simulink model "AvonGasTurbineDgTwin"  (R2024b)
settings: Solver=VariableStepAuto  StartTime=0  StopTime=7200  FixedStep=1  RelTol=1e-3  EnableMultiTasking=on
InitFcn:
  | warning off
undefined symbols (not defined in the file or in its folder): ENV_ambient_moisture_pct, ENV_comp_inlet_press_kPa, ENV_comp_inlet_temp_C, ENV_FG_pressure_kPa, ENV_FG_temp_C
libraries: slpidlib x3, simulink x2
(part 2 of 3)

== system AvonGasTurbineDgTwin/FAULT_06_IGVStuck ==
  IGV Pos : Inport
  FAULT_06_multiplier : FromWorkspace  VariableName=FAULT_06_multiplier  SampleTime=-1
  Mux : Mux  Inputs=2
  Product : Product
  Scope{,1..3} (4 alike) : Scope  Commented=on
  Out1 : Outport
  wires:
  FAULT_06_multiplier/1 -> Product/1, Scope/1
  IGV Pos/1 -> Scope1/1, Mux/2, Product/2
  Product/1 -> Mux/1, Scope2/1, Out1/1
  Mux/1 -> Scope3/1

== system AvonGasTurbineDgTwin/FAULT_15_FuelPressReg ==
  In1 : Inport
  FAULT_15_multiplier : FromWorkspace  VariableName=FAULT_15_multiplier  SampleTime=-1
  Mux : Mux  Inputs=2
  Product : Product
  Scope{,1..3} (4 alike) : Scope  Commented=on
  Out1 : Outport
  wires:
  FAULT_15_multiplier/1 -> Product/1, Scope/1
  In1/1 -> Scope1/1, Mux/2, Product/2
  Product/1 -> Mux/1, Scope2/1, Out1/1
  Mux/1 -> Scope3/1

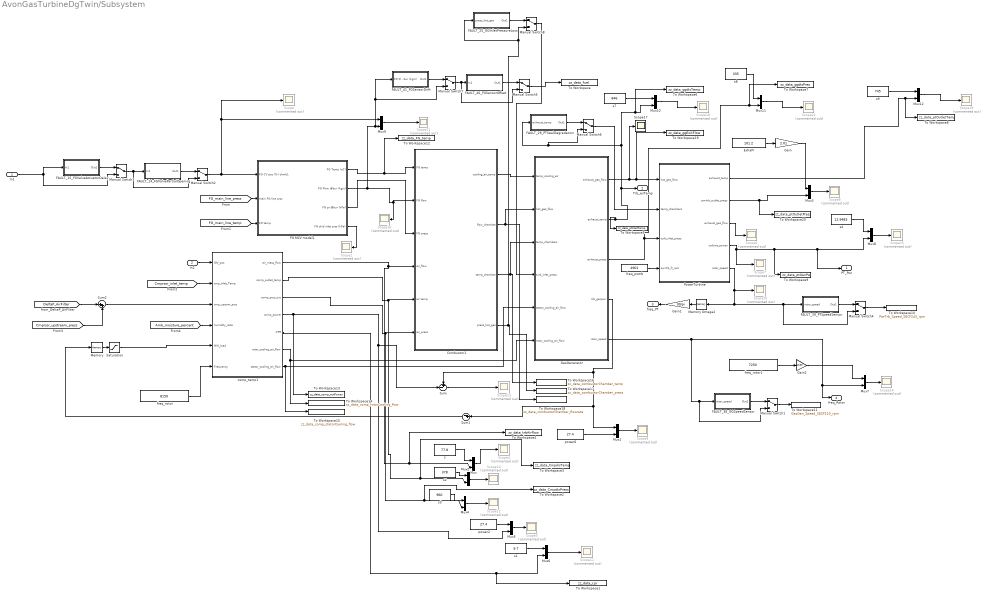
== system AvonGasTurbineDgTwin/Subsystem ==
  In1 : Inport
  In2 : Inport  Port=2
  Combustor1 : Subsystem
  ExhaPr : Constant  Value=101.2
  FAULT_14_FGValvePartialOpening : Subsystem
  FAULT_15_FGValveActuatorDelay : Subsystem
  FAULT_25_GGInletPressureLoss : Subsystem
  FAULT_29_PTSealDegradation : Subsystem
  FAULT_38_GGSpeedSensor : Subsystem
  FAULT_39_PTSpeedSensor : Subsystem
  FAULT_40_FGSensorOffset : Subsystem
  FAULT_41_FGSensorDrift : Subsystem
  FG MCV model1 : Subsystem
  Gain : Gain  Gain=2.01
  Gain1 : Gain  Gain=30/pi
  Gain2 : Gain  Gain=pi/30
  GasGenerator : Subsystem
  Manual Switch{1..8} (8 alike) : ManualSwitch
  Memory : Memory  InitialCondition=28.945
  Memory Omega2 : Memory  InitialCondition=pi/30*4901
  Mux{,1..12} (13 alike) : Mux  Inputs=2
  PowerTurbine : Subsystem
  Saturation : Saturate  UpperLimit=40  LowerLimit=1
  Scope{,2..4,6..16,18..22} (20 alike) : Scope  Commented=on
  Scope17 : Scope
  Sum : Sum  Inputs=+-|
  Sum1 : Sum  Inputs=-+|
  Sum2 : Sum  Inputs=|++
  To Workspace : ToWorkspace  VariableName=zz_data_fuel  SampleTime=0.2
  To Workspace1 : ToWorkspace  VariableName=zz_data_cpr  SampleTime=0.2
  To Workspace10 : ToWorkspace  VariableName=PwrTrb_Speed_SECF243_rpm  SampleTime=0.2
  To Workspace11 : ToWorkspace  VariableName=GasGen_Speed_SECF210_rpm  SampleTime=0.2
  To Workspace12 : ToWorkspace  VariableName=zz_data_FG_temp  SampleTime=0.2
  To Workspace13 : ToWorkspace  VariableName=zz_data_comp_outPower  SampleTime=0.2
  To Workspace14 : ToWorkspace  VariableName=zz_data_comp_rotorCooling_flow  SampleTime=0.2
  To Workspace15 : ToWorkspace  VariableName=zz_data_comp_statorCooling_flow  SampleTime=0.2
  To Workspace16 : ToWorkspace  VariableName=zz_data_combustorChamber_temp  SampleTime=0.2
  To Workspace17 : ToWorkspace  VariableName=zz_data_combustorChamber_press  SampleTime=0.2
  To Workspace18 : ToWorkspace  VariableName=zz_data_combustorChamber_flowrate  SampleTime=0.2
  To Workspace19 : ToWorkspace  VariableName=zz_data_ggExitFlow  SampleTime=0.2
  To Workspace2 : ToWorkspace  VariableName=zz_data_CmpdisPress  SampleTime=0.2
  To Workspace20 : ToWorkspace  VariableName=zz_data_ptOutletPress  SampleTime=0.2
  To Workspace3 : ToWorkspace  VariableName=zz_data_CmpdisTemp  SampleTime=0.2
  To Workspace4 : ToWorkspace  VariableName=zz_data_trbAirflow  SampleTime=0.2
  To Workspace5 : ToWorkspace  VariableName=zz_data_ptInletTemp  SampleTime=0.2
  To Workspace6 : ToWorkspace  VariableName=zz_data_ggdisTemp  SampleTime=0.2
  To Workspace7 : ToWorkspace  VariableName=zz_data_ggdisPres  SampleTime=0.2
  To Workspace8 : ToWorkspace  VariableName=zz_data_ptOutletTemp  SampleTime=0.2
  To Workspace9 : ToWorkspace  VariableName=zz_data_ptGenPw  SampleTime=0.2
  comp_temp1 : Subsystem
  freq_pwtrb : Constant  Value=4901
  freq_rotor : Constant  Value=8150
  freq_rotor1 : Constant  Value=7250
  power2 : Constant  Value=27.4
  power6 : Constant  Value=27.4
  s : Constant  Value=77.8
  s1 : Constant  Value=9.7
  s2 : Constant  Value=378
  s3 : Constant  Value=960
  s4 : Constant  Value=12.9483
  s7 : Constant  Value=846
  s8 : Constant  Value=335
  s9 : Constant  Value=745
  PT_Pwr : Outport
  Trb_exTemp : Outport  Port=2
  freq_PT : Outport  Port=3
  freq_Rotor : Outport  Port=4
  wires:
  Gain1/1 -> freq_PT/1
  GasGenerator/2(exhaust_temp) -> To Workspace5/1, Trb_exTemp/1, Manual Switch6/2, FAULT_29_PTSealDegradation/1(exhaust_temp), To Workspace6/1, Mux10/2
  [Amb_moisture_percent] -> comp_temp1/4(humidity_ratio)
  freq_rotor/1 -> comp_temp1/6(Frequency)
  In2/1 -> comp_temp1/1(IGV_pos)
  PowerTurbine/3(exhaust_gas_flow) -> Scope6/1
  Memory/1 -> Saturation/1
  comp_temp1/3(comp_prss_out) -> To Workspace2/1, Mux4/2, Combustor1/6(air_press)
  FG MCV model1/2(FG Flow @bur (kg/s)) -> Manual Switch7/2, FAULT_41_FGSensorDrift/1(FG Flow @bur (kg/s)), Mux9/2, Scope16/1, Combustor1/2(FG flow)
  Combustor1/2(flow_chamber) -> To Workspace18/1, GasGenerator/2(hot_gas_flow)
  comp_temp1/4(comp_power) -> To Workspace13/1, Mux5/2, Sum/2
  Mux1/1 -> Scope9/1
  Mux6/1 -> Scope11/1
  comp_temp1/5(CPR) -> To Workspace1/1, Mux6/2
  Mux4/1 -> Scope12/1
  FG MCV model1/1(FG Temp (oC)) -> To Workspace12/1, Combustor1/1(FG temp)
  Mux2/1 -> Scope10/1
  [FG_main_line_press] -> FG MCV model1/2(main FG line prss)
  ExhaPr/1 -> Gain/1
  Combustor1/1(cooling_air_temp) -> GasGenerator/1(temp_cooling_air)
  FG MCV model1/3(FG pr @bur (kPa)) -> Combustor1/3(FG press)
  GasGenerator/3(exhaust_press) -> To Workspace7/1, Mux11/2, PowerTurbine/3(turb_inlet_press)
  Combustor1/3(temp_chamber) -> To Workspace16/1, GasGenerator/3(temp_chambers)
  FG MCV model1/4(FG skid inlet prss (kPa)) -> Scope2/1
  GasGenerator/1(exhaust_gas_flow) -> Scope17/1, To Workspace19/1, PowerTurbine/1(hot_gas_flow)
  PowerTurbine/2(pwrtrb_outlet_press) -> To Workspace20/1, Mux3/2
  power6/1 -> Mux1/2
  Gain/1 -> Mux3/1
  Mux3/1 -> Scope8/1
  comp_temp1/1(air_mass_flow) -> To Workspace4/1, Mux/2, Combustor1/4(air_flow)
  PowerTurbine/1(exhaust_temp) -> To Workspace8/1, Mux12/2
  comp_temp1/2(comp_outlet_temp) -> To Workspace3/1, Mux2/2, Combustor1/5(air temp)
  Mux8/1 -> Scope15/1
  Mux7/1 -> Scope14/1
  In1/1 -> FAULT_15_FGValveActuatorDelay/1(In1), Manual Switch3/2
  PowerTurbine/4(turbine_power) -> To Workspace9/1, PT_Pwr/1, Mux8/2, Scope7/1
  comp_temp1/7(stator_cooling_air_flow) -> GasGenerator/5(stator_cooling_air_flow), To Workspace15/1
  [Cmprssr_inlet_temp] -> comp_temp1/2(cmp_Inlet_Temp)
  Mux11/1 -> Scope22/1
  s2/1 -> Mux2/1
  Sum1/1 -> Memory/1
  Mux9/1 -> Scope21/1
  Mux/1 -> Scope4/1
  s/1 -> Mux/1
  s7/1 -> Mux10/1
  s1/1 -> Mux6/1
  Mux10/1 -> Scope18/1
  Mux5/1 -> Scope3/1
  Sum/1 -> Scope13/1
  GasGenerator/5(rotor_speed) -> Manual Switch1/2, FAULT_38_GGSpeedSensor/1(rotor_speed), freq_Rotor/1, Mux7/2
  comp_temp1/6(rotor_cooling_air_flow) -> GasGenerator/6(rotor_cooling_air_flow), To Workspace14/1
  s3/1 -> Mux4/1
  freq_pwtrb/1 -> PowerTurbine/4(pwrtrb_fr_rpm)
  power2/1 -> Mux5/1
  PowerTurbine/5(rotor_speed) -> Manual Switch4/2, FAULT_39_PTSpeedSensor/1(rotor_speed), Memory Omega2/1, Scope20/1
  Gain2/1 -> Mux7/1
  Saturation/1 -> comp_temp1/5(MW_load)
  Memory Omega2/1 -> Gain1/1
  freq_rotor1/1 -> Gain2/1
  GasGenerator/4(trb_genpwr) -> Sum/1, Sum1/2, Mux1/1
  s4/1 -> Mux8/1
  s9/1 -> Mux12/1
  s8/1 -> Mux11/1
  Mux12/1 -> Scope19/1
  [FG_main_line_temp] -> FG MCV model1/3(FG temp.)
  FAULT_41_FGSensorDrift/1(Out1) -> Manual Switch7/1
  FAULT_14_FGValvePartialOpening/1(Out1) -> Manual Switch2/1
  FAULT_15_FGValveActuatorDelay/1(Out1) -> Manual Switch3/1
  Manual Switch3/1 -> Manual Switch2/2, FAULT_14_FGValvePartialOpening/1(In1)
  Manual Switch2/1 -> Mux9/1, Scope/1, FG MCV model1/1(FG CV pos (%) chmb1)
  FAULT_38_GGSpeedSensor/1(Out1) -> Manual Switch1/1
  Manual Switch1/1 -> To Workspace11/1
  FAULT_39_PTSpeedSensor/1(Out1) -> Manual Switch4/1
  Manual Switch4/1 -> To Workspace10/1
  FAULT_40_FGSensorOffset/1(Out1) -> Manual Switch5/1
  Manual Switch7/1 -> Manual Switch5/2, FAULT_40_FGSensorOffset/1(In1)
  Manual Switch5/1 -> To Workspace/1
  [DeltaP_AirFilter] -> Sum2/1
  [Cmprssr_upstream_press] -> Sum2/2
  Sum2/1 -> comp_temp1/3(cmp_upstrm_prss)
  FAULT_29_PTSealDegradation/1(Out1) -> Manual Switch6/1
  Manual Switch6/1 -> PowerTurbine/2(temp_chambers)
  Combustor1/4(press_hot_gas) -> Manual Switch8/2, FAULT_25_GGInletPressureLoss/1(press_hot_gas), To Workspace17/1
  FAULT_25_GGInletPressureLoss/1(Out1) -> Manual Switch8/1
  Manual Switch8/1 -> GasGenerator/4(turb_inlet_press)

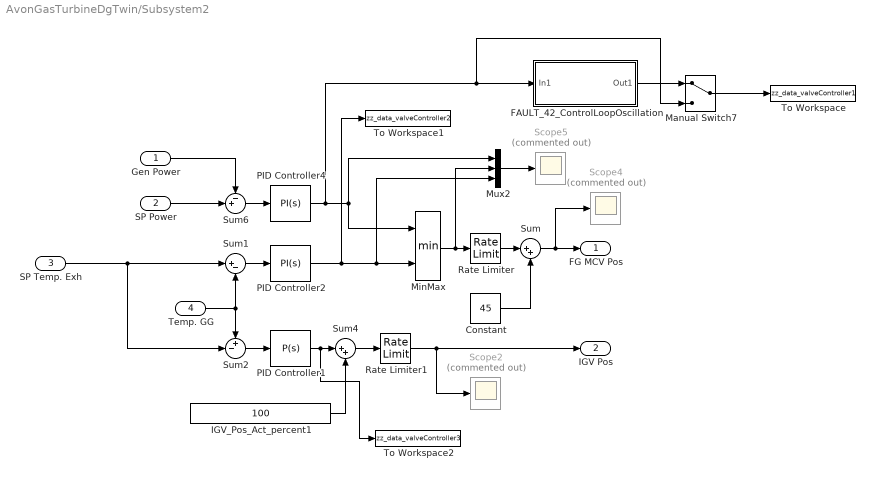
== system AvonGasTurbineDgTwin/Subsystem2 ==
  Gen Power : Inport
  SP Power : Inport  Port=2
  SP Temp. Exh : Inport  Port=3
  Temp. GG : Inport  Port=4
  Constant : Constant  Value=45
  FAULT_42_ControlLoopOscillation : Subsystem
  IGV_Pos_Act_percent1 : Constant  Value=100
  Manual Switch7 : ManualSwitch
  MinMax : MinMax  Inputs=2
  Mux2 : Mux  Inputs=3
  PID Controller1 : slpidlib/PID Controller  Controller=P  Form=Ideal  TimeDomain=Continuous-time  UseExternalTs=off  SampleTime=-1  IntegratorMethod=Forward Euler  FilterMethod=Forward Euler  ControllerParametersSource=internal  P=0.1  I=0.180070827922895  UseKiTs=off  D=0  UseExternalDerivativeSource=off  N=100  UseFilter=on  TunerSelectOption=Transfer Function Based (PID Tuner App)  InitialConditionSource=internal  InitialConditionForIntegrator=0  InitialConditionForFilter=0  DifferentiatorICPrevScaledInput=0  ExternalReset=none  TrackingMode=off  Kt=1  LimitOutput=on  SatLimitsSource=internal  UpperSaturationLimit=15  LowerSaturationLimit=-100  LinearizeAsGain=on  AntiWindupMode=back-calculation  Kb=0.2  LimitIntegrator=off  UpperIntegratorSaturationLimit=inf  LowerIntegratorSaturationLimit=-inf  POutMin=[]  POutMax=[]  IOutMin=[]  IOutMax=[]  DOutMin=[]  DOutMax=[]  NOutMin=[]  NOutMax=[]  SumOutMin=[]  SumOutMax=[]  SaturationOutMin=[]  SaturationOutMax=[]  PParamMin=[]  PParamMax=[]  IParamMin=[]  IParamMax=[]  DParamMin=[]  DParamMax=[]  NParamMin=[]  NParamMax=[]  KbParamMin=[]  KbParamMax=[]  KtParamMin=[]  KtParamMax=[]  KbOutMin=[]  KbOutMax=[]  KtOutMin=[]  KtOutMax=[]  IntegratorOutMin=[]  IntegratorOutMax=[]  FilterOutMin=[]  FilterOutMax=[]  SumI1OutMin=[]  SumI1OutMax=[]  SumI2OutMin=[]  SumI2OutMax=[]  SumI3OutMin=[]  SumI3OutMax=[]  SumI4OutMin=[]  SumI4OutMax=[]  SumDOutMin=[]  SumDOutMax=[]  DifferentiatorOutMin=[]  DifferentiatorOutMax=[]  FilterDiffOutCoefMin=[]  FilterDiffOutCoefMax=[]  ReciprocalOutMin=[]  ReciprocalOutMax=[]  SumDenOutMin=[]  SumDenOutMax=[]  SumNumOutMin=[]  SumNumOutMax=[]  DivideOutMin=[]  DivideOutMax=[]  UdiffTsProdOutMin=[]  UdiffTsProdOutMax=[]  NTsProdOutMin=[]  NTsProdOutMax=[]  UintegralTsProdOutMin=[]  UintegralTsProdOutMax=[]  UngainTsProdOutMin=[]  UngainTsProdOutMax=[]  ClampingZeroOutDataTypeStr=Inherit: Inherit via back propagation  ClampingZeroOutMin=[]  ClampingZeroOutMax=[]  FilterDenConstantOutDataTypeStr=Inherit: Inherit via back propagation  FilterDenConstantOutMin=[]  FilterDenConstantOutMax=[]  PCopyOutDataTypeStr=Inherit: Inherit via back propagation  PCopyOutMin=[]  PCopyOutMax=[]  NCopyOutDataTypeStr=Inherit: Inherit via back propagation  NCopyOutMin=[]  NCopyOutMax=[]  IntegratorContinuousStateAttributes=''  IntegratorStateMustResolveToSignalObject=off  IntegratorRTWStateStorageClass=Auto  FilterContinuousStateAttributes=''  FilterStateMustResolveToSignalObject=off  FilterRTWStateStorageClass=Auto  ParallelPVariant=InternalParameters  IdealPVariant=Disabled  IVariant=Disabled  DVariant=Disabled  IntegratorVariant=Disabled  SatVariant=Enabled  AWVariant=Disabled  PCopyVariant=Disabled  TRVariant=Disabled  FdbkBlocksVariant=Forward  IdealPFdbkVariant=Disabled  SatFdbkVariant=Disabled  DerivativeFilterVariant=Disabled  NVariant=Disabled  NCopyVariant=Disabled_SignalSpec  FilterICVariant=Disabled  IntegratorICVariant=Disabled  ExternalResetVariant=Disabled  TRSumVariant=Passthrough  SumFdbkVariant=Disabled  SumVariant=Passthrough_P  TsampFilterVariant=InternalTs  TsampNgainVariant=Passthrough  TsampIntegralVariant=Disabled_SignalSpec  ExternalSaturationOutDataTypeStr=Inherit: Same as second input  DerivativeSourceVariant=Disabled  PreIntVariant=InternalPreInt
  PID Controller2 : slpidlib/PID Controller  Controller=PI  Form=Ideal  TimeDomain=Continuous-time  UseExternalTs=off  SampleTime=-1  IntegratorMethod=Forward Euler  FilterMethod=Forward Euler  ControllerParametersSource=internal  P=0.02  I=0.1  UseKiTs=off  D=0  UseExternalDerivativeSource=off  N=100  UseFilter=on  TunerSelectOption=Transfer Function Based (PID Tuner App)  InitialConditionSource=internal  InitialConditionForIntegrator=20  InitialConditionForFilter=0  DifferentiatorICPrevScaledInput=0  ExternalReset=none  TrackingMode=off  Kt=1  LimitOutput=on  SatLimitsSource=internal  UpperSaturationLimit=45  LowerSaturationLimit=-45  LinearizeAsGain=on  AntiWindupMode=back-calculation  Kb=0.2  LimitIntegrator=off  UpperIntegratorSaturationLimit=inf  LowerIntegratorSaturationLimit=-inf  POutMin=[]  POutMax=[]  IOutMin=[]  IOutMax=[]  DOutMin=[]  DOutMax=[]  NOutMin=[]  NOutMax=[]  SumOutMin=[]  SumOutMax=[]  SaturationOutMin=[]  SaturationOutMax=[]  PParamMin=[]  PParamMax=[]  IParamMin=[]  IParamMax=[]  DParamMin=[]  DParamMax=[]  NParamMin=[]  NParamMax=[]  KbParamMin=[]  KbParamMax=[]  KtParamMin=[]  KtParamMax=[]  KbOutMin=[]  KbOutMax=[]  KtOutMin=[]  KtOutMax=[]  IntegratorOutMin=[]  IntegratorOutMax=[]  FilterOutMin=[]  FilterOutMax=[]  SumI1OutMin=[]  SumI1OutMax=[]  SumI2OutMin=[]  SumI2OutMax=[]  SumI3OutMin=[]  SumI3OutMax=[]  SumI4OutMin=[]  SumI4OutMax=[]  SumDOutMin=[]  SumDOutMax=[]  DifferentiatorOutMin=[]  DifferentiatorOutMax=[]  FilterDiffOutCoefMin=[]  FilterDiffOutCoefMax=[]  ReciprocalOutMin=[]  ReciprocalOutMax=[]  SumDenOutMin=[]  SumDenOutMax=[]  SumNumOutMin=[]  SumNumOutMax=[]  DivideOutMin=[]  DivideOutMax=[]  UdiffTsProdOutMin=[]  UdiffTsProdOutMax=[]  NTsProdOutMin=[]  NTsProdOutMax=[]  UintegralTsProdOutMin=[]  UintegralTsProdOutMax=[]  UngainTsProdOutMin=[]  UngainTsProdOutMax=[]  ClampingZeroOutDataTypeStr=Inherit: Inherit via back propagation  ClampingZeroOutMin=[]  ClampingZeroOutMax=[]  FilterDenConstantOutDataTypeStr=Inherit: Inherit via back propagation  FilterDenConstantOutMin=[]  FilterDenConstantOutMax=[]  PCopyOutDataTypeStr=Inherit: Inherit via back propagation  PCopyOutMin=[]  PCopyOutMax=[]  NCopyOutDataTypeStr=Inherit: Inherit via back propagation  NCopyOutMin=[]  NCopyOutMax=[]  IntegratorContinuousStateAttributes=''  IntegratorStateMustResolveToSignalObject=off  IntegratorRTWStateStorageClass=Auto  FilterContinuousStateAttributes=''  FilterStateMustResolveToSignalObject=off  FilterRTWStateStorageClass=Auto  ParallelPVariant=Passthrough  IdealPVariant=InternalParameters  IVariant=InternalParameters  DVariant=Disabled  IntegratorVariant=Continuous  SatVariant=Enabled  AWVariant=BackCalculation  PCopyVariant=Disabled  TRVariant=Disabled  FdbkBlocksVariant=Forward  IdealPFdbkVariant=Disabled  SatFdbkVariant=Disabled  DerivativeFilterVariant=Disabled  NVariant=Disabled  NCopyVariant=Disabled_SignalSpec  FilterICVariant=Disabled  IntegratorICVariant=InternalICs  ExternalResetVariant=Disabled  TRSumVariant=Passthrough  SumFdbkVariant=Disabled  SumVariant=Sum_PI  TsampFilterVariant=InternalTs  TsampNgainVariant=Passthrough  TsampIntegralVariant=Disabled_SignalSpec  ExternalSaturationOutDataTypeStr=Inherit: Same as second input  DerivativeSourceVariant=Disabled  PreIntVariant=InternalPreInt
  PID Controller4 : slpidlib/PID Controller  Controller=PI  Form=Ideal  TimeDomain=Continuous-time  UseExternalTs=off  SampleTime=-1  IntegratorMethod=Forward Euler  FilterMethod=Forward Euler  ControllerParametersSource=internal  P=0.17  I=0.2  UseKiTs=off  D=0  UseExternalDerivativeSource=off  N=100  UseFilter=on  TunerSelectOption=Transfer Function Based (PID Tuner App)  InitialConditionSource=internal  InitialConditionForIntegrator=0  InitialConditionForFilter=0  DifferentiatorICPrevScaledInput=0  ExternalReset=none  TrackingMode=off  Kt=1  LimitOutput=on  SatLimitsSource=internal  UpperSaturationLimit=60  LowerSaturationLimit=-30  LinearizeAsGain=on  AntiWindupMode=back-calculation  Kb=0.2  LimitIntegrator=off  UpperIntegratorSaturationLimit=inf  LowerIntegratorSaturationLimit=-inf  POutMin=[]  POutMax=[]  IOutMin=[]  IOutMax=[]  DOutMin=[]  DOutMax=[]  NOutMin=[]  NOutMax=[]  SumOutMin=[]  SumOutMax=[]  SaturationOutMin=[]  SaturationOutMax=[]  PParamMin=[]  PParamMax=[]  IParamMin=[]  IParamMax=[]  DParamMin=[]  DParamMax=[]  NParamMin=[]  NParamMax=[]  KbParamMin=[]  KbParamMax=[]  KtParamMin=[]  KtParamMax=[]  KbOutMin=[]  KbOutMax=[]  KtOutMin=[]  KtOutMax=[]  IntegratorOutMin=[]  IntegratorOutMax=[]  FilterOutMin=[]  FilterOutMax=[]  SumI1OutMin=[]  SumI1OutMax=[]  SumI2OutMin=[]  SumI2OutMax=[]  SumI3OutMin=[]  SumI3OutMax=[]  SumI4OutMin=[]  SumI4OutMax=[]  SumDOutMin=[]  SumDOutMax=[]  DifferentiatorOutMin=[]  DifferentiatorOutMax=[]  FilterDiffOutCoefMin=[]  FilterDiffOutCoefMax=[]  ReciprocalOutMin=[]  ReciprocalOutMax=[]  SumDenOutMin=[]  SumDenOutMax=[]  SumNumOutMin=[]  SumNumOutMax=[]  DivideOutMin=[]  DivideOutMax=[]  UdiffTsProdOutMin=[]  UdiffTsProdOutMax=[]  NTsProdOutMin=[]  NTsProdOutMax=[]  UintegralTsProdOutMin=[]  UintegralTsProdOutMax=[]  UngainTsProdOutMin=[]  UngainTsProdOutMax=[]  ClampingZeroOutDataTypeStr=Inherit: Inherit via back propagation  ClampingZeroOutMin=[]  ClampingZeroOutMax=[]  FilterDenConstantOutDataTypeStr=Inherit: Inherit via back propagation  FilterDenConstantOutMin=[]  FilterDenConstantOutMax=[]  PCopyOutDataTypeStr=Inherit: Inherit via back propagation  PCopyOutMin=[]  PCopyOutMax=[]  NCopyOutDataTypeStr=Inherit: Inherit via back propagation  NCopyOutMin=[]  NCopyOutMax=[]  IntegratorContinuousStateAttributes=''  IntegratorStateMustResolveToSignalObject=off  IntegratorRTWStateStorageClass=Auto  FilterContinuousStateAttributes=''  FilterStateMustResolveToSignalObject=off  FilterRTWStateStorageClass=Auto  ParallelPVariant=Passthrough  IdealPVariant=InternalParameters  IVariant=InternalParameters  DVariant=Disabled  IntegratorVariant=Continuous  SatVariant=Enabled  AWVariant=BackCalculation  PCopyVariant=Disabled  TRVariant=Disabled  FdbkBlocksVariant=Forward  IdealPFdbkVariant=Disabled  SatFdbkVariant=Disabled  DerivativeFilterVariant=Disabled  NVariant=Disabled  NCopyVariant=Disabled_SignalSpec  FilterICVariant=Disabled  IntegratorICVariant=InternalICs  ExternalResetVariant=Disabled  TRSumVariant=Passthrough  SumFdbkVariant=Disabled  SumVariant=Sum_PI  TsampFilterVariant=InternalTs  TsampNgainVariant=Passthrough  TsampIntegralVariant=Disabled_SignalSpec  ExternalSaturationOutDataTypeStr=Inherit: Same as second input  DerivativeSourceVariant=Disabled  PreIntVariant=InternalPreInt
  Rate Limiter : RateLimiter  RisingSlewLimit=0.1  FallingSlewLimit=-0.1  SampleTimeMode=inherited  InitialCondition=45
  Rate Limiter1 : RateLimiter  RisingSlewLimit=0.1  FallingSlewLimit=-0.1  SampleTimeMode=inherited  InitialCondition=45
  Scope2 : Scope  Commented=on
  Scope4 : Scope  Commented=on
  Scope5 : Scope  Commented=on
  Sum : Sum  Inputs=|++
  Sum1 : Sum  Inputs=|+-
  Sum2 : Sum  Inputs=+-|
  Sum4 : Sum  Inputs=|++
  Sum6 : Sum  Inputs=-+|
  To Workspace : ToWorkspace  VariableName=zz_data_valveController1  SampleTime=0.2
  To Workspace1 : ToWorkspace  VariableName=zz_data_valveController2  SampleTime=0.2
  To Workspace2 : ToWorkspace  VariableName=zz_data_valveController3  SampleTime=0.2
  FG MCV Pos : Outport
  IGV Pos : Outport  Port=2
  wires:
  Gen Power/1 -> Sum6/1
  MinMax/1 -> Mux2/2, Rate Limiter/1
  Mux2/1 -> Scope5/1
  Sum6/1 -> PID Controller4/1
  PID Controller4/1 -> Manual Switch7/2, FAULT_42_ControlLoopOscillation/1(In1), Mux2/1, MinMax/1
  SP Temp. Exh/1 -> Sum2/2, Sum1/1
  Temp. GG/1 -> Sum2/1, Sum1/2
  Sum/1 -> FG MCV Pos/1, Scope4/1
  Constant/1 -> Sum/2
  Sum2/1 -> PID Controller1/1
  IGV_Pos_Act_percent1/1 -> Sum4/2
  PID Controller1/1 -> To Workspace2/1, Sum4/1
  Sum4/1 -> Rate Limiter1/1
  PID Controller2/1 -> MinMax/2, Mux2/3, To Workspace1/1
  Rate Limiter1/1 -> IGV Pos/1, Scope2/1
  Rate Limiter/1 -> Sum/1
  SP Power/1 -> Sum6/2
  Sum1/1 -> PID Controller2/1
  FAULT_42_ControlLoopOscillation/1(Out1) -> Manual Switch7/1
  Manual Switch7/1 -> To Workspace/1

== system AvonGasTurbineDgTwin/Subsystem/Combustor1 ==
  FG temp : Inport
  FG flow : Inport  Port=2
  FG press : Inport  Port=3
  air_flow : Inport  Port=4
  air temp : Inport  Port=5
  air_press : Inport  Port=6
  FAULT_16_CombLinerDamage : Subsystem
  FAULT_17_FuelNozzleClogging : Subsystem
  FAULT_18_CombustionFlameOscillation : Subsystem
  FAULT_19_CombustionInstability : Subsystem
  FAULT_20_HotGasPathTempIncrease : Subsystem
  Manual Switch{1..4,7} (5 alike) : ManualSwitch
  Scope{1..4} (4 alike) : Scope
  combustion chamber 1 : Subsystem
  cooling_air_temp : Outport
  flow_chamber : Outport  Port=2
  temp_chamber : Outport  Port=3
  press_hot_gas : Outport  Port=4
  wires:
  FG press/1 -> combustion chamber 1/2(FG press)
  FG temp/1 -> combustion chamber 1/3(FG temp)
  air_press/1 -> combustion chamber 1/6(air_press)
  air temp/1 -> Scope2/1, cooling_air_temp/1, combustion chamber 1/5(air_temp)
  combustion chamber 1/2(flow) -> Scope3/1, flow_chamber/1
  combustion chamber 1/3(Gas_press) -> press_hot_gas/1
  FAULT_16_CombLinerDamage/1(Out1) -> Manual Switch7/1
  Manual Switch7/1 -> Scope4/1, combustion chamber 1/4(air flow)
  air_flow/1 -> Manual Switch7/2, FAULT_16_CombLinerDamage/1(air_flow)
  FAULT_17_FuelNozzleClogging/1(Out1) -> Manual Switch1/1
  FAULT_20_HotGasPathTempIncrease/1(Out1) -> Manual Switch2/1
  Manual Switch1/1 -> combustion chamber 1/1(Fg flow)
  FG flow/1 -> Manual Switch1/2, FAULT_17_FuelNozzleClogging/1(FG flow)
  FAULT_18_CombustionFlameOscillation/1(Out1) -> Manual Switch3/1
  combustion chamber 1/1(temp chamber 1) -> Manual Switch3/2, FAULT_18_CombustionFlameOscillation/1(temp chamber 1)
  FAULT_19_CombustionInstability/1(Out1) -> Manual Switch4/1
  Manual Switch3/1 -> Manual Switch4/2, FAULT_19_CombustionInstability/1(In1)
  Manual Switch4/1 -> Manual Switch2/2, FAULT_20_HotGasPathTempIncrease/1(In1)
  Manual Switch2/1 -> Scope1/1, temp_chamber/1

== system AvonGasTurbineDgTwin/Subsystem/FAULT_14_FGValvePartialOpening ==
  In1 : Inport
  FAULT_14_multiplier : FromWorkspace  VariableName=FAULT_14_multiplier  SampleTime=-1
  Mux : Mux  Inputs=2
  Product : Product
  Scope{,1..3} (4 alike) : Scope  Commented=on
  Out1 : Outport
  wires:
  FAULT_14_multiplier/1 -> Product/1, Scope/1
  In1/1 -> Scope1/1, Mux/2, Product/2
  Product/1 -> Mux/1, Scope2/1, Out1/1
  Mux/1 -> Scope3/1

== system AvonGasTurbineDgTwin/Subsystem/FAULT_15_FGValveActuatorDelay ==
  In1 : Inport
  FAULT_15_multiplier : FromWorkspace  VariableName=FAULT_15_multiplier  SampleTime=-1
  Mux : Mux  Inputs=2
  Product : Product
  Scope{,1..3} (4 alike) : Scope  Commented=on
  Out1 : Outport
  wires:
  FAULT_15_multiplier/1 -> Product/1, Scope/1
  In1/1 -> Scope1/1, Mux/2, Product/2
  Product/1 -> Mux/1, Scope2/1, Out1/1
  Mux/1 -> Scope3/1

== system AvonGasTurbineDgTwin/Subsystem/FAULT_25_GGInletPressureLoss ==
  press_hot_gas : Inport
  FAULT_25_multiplier : FromWorkspace  VariableName=FAULT_25_multiplier  SampleTime=-1
  Mux : Mux  Inputs=2
  Product : Product
  Scope{,1..3} (4 alike) : Scope  Commented=on
  Out1 : Outport
  wires:
  FAULT_25_multiplier/1 -> Product/1, Scope/1
  press_hot_gas/1 -> Scope1/1, Mux/2, Product/2
  Product/1 -> Mux/1, Scope2/1, Out1/1
  Mux/1 -> Scope3/1

== system AvonGasTurbineDgTwin/Subsystem/FAULT_29_PTSealDegradation ==
  exhaust_temp : Inport
  FAULT_29_multiplier : FromWorkspace  VariableName=FAULT_29_multiplier  SampleTime=-1
  Mux : Mux  Inputs=2
  Product : Product
  Scope{,1..3} (4 alike) : Scope  Commented=on
  Out1 : Outport
  wires:
  FAULT_29_multiplier/1 -> Product/1, Scope/1
  exhaust_temp/1 -> Scope1/1, Mux/2, Product/2
  Product/1 -> Mux/1, Scope2/1, Out1/1
  Mux/1 -> Scope3/1

== system AvonGasTurbineDgTwin/Subsystem/FAULT_38_GGSpeedSensor ==
  rotor_speed : Inport
  FAULT_38_multiplier : FromWorkspace  VariableName=FAULT_38_multiplier  SampleTime=-1
  Mux : Mux  Inputs=2
  Product : Product
  Scope{,1..3} (4 alike) : Scope  Commented=on
  Out1 : Outport
  wires:
  FAULT_38_multiplier/1 -> Product/1, Scope/1
  rotor_speed/1 -> Scope1/1, Mux/2, Product/2
  Product/1 -> Mux/1, Scope2/1, Out1/1
  Mux/1 -> Scope3/1

== system AvonGasTurbineDgTwin/Subsystem/FAULT_39_PTSpeedSensor ==
  rotor_speed : Inport
  FAULT_39_multiplier : FromWorkspace  VariableName=FAULT_39_multiplier  SampleTime=-1
  Mux : Mux  Inputs=2
  Product : Product
  Scope{,1..3} (4 alike) : Scope  Commented=on
  Out1 : Outport
  wires:
  FAULT_39_multiplier/1 -> Product/1, Scope/1
  rotor_speed/1 -> Scope1/1, Mux/2, Product/2
  Product/1 -> Mux/1, Scope2/1, Out1/1
  Mux/1 -> Scope3/1

== system AvonGasTurbineDgTwin/Subsystem/FAULT_40_FGSensorOffset ==
  In1 : Inport
  FAULT_40_multiplier : FromWorkspace  VariableName=FAULT_40_multiplier  SampleTime=-1
  Mux : Mux  Inputs=2
  Product : Product
  Scope{,1..3} (4 alike) : Scope  Commented=on
  Out1 : Outport
  wires:
  FAULT_40_multiplier/1 -> Product/1, Scope/1
  In1/1 -> Scope1/1, Mux/2, Product/2
  Product/1 -> Mux/1, Scope2/1, Out1/1
  Mux/1 -> Scope3/1

== system AvonGasTurbineDgTwin/Subsystem/FAULT_41_FGSensorDrift ==
  FG Flow @bur (kg/s) : Inport
  FAULT_41_multiplier : FromWorkspace  VariableName=FAULT_41_multiplier  SampleTime=-1
  Mux : Mux  Inputs=2
  Product : Product
  Scope{,1..3} (4 alike) : Scope  Commented=on
  Out1 : Outport
  wires:
  FAULT_41_multiplier/1 -> Product/1, Scope/1
  FG Flow @bur (kg/s)/1 -> Scope1/1, Mux/2, Product/2
  Product/1 -> Mux/1, Scope2/1, Out1/1
  Mux/1 -> Scope3/1

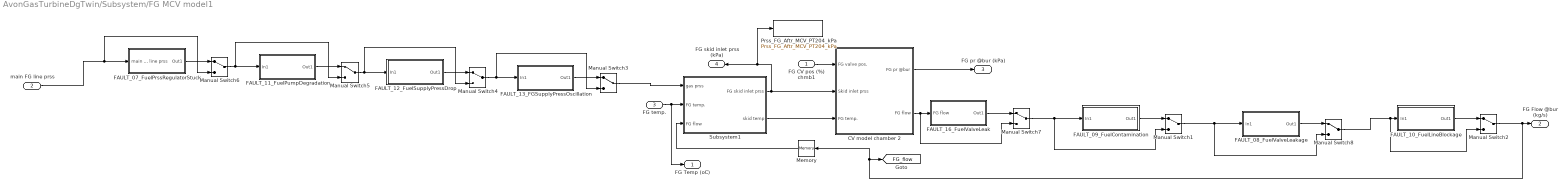
== system AvonGasTurbineDgTwin/Subsystem/FG MCV model1 ==
  FG CV pos (%) chmb1 : Inport
  main FG line prss : Inport  Port=2
  FG temp. : Inport  Port=3
  " Memory " : Memory  InitialCondition=1.9
  CV model chamber 2 : Subsystem
  FAULT_07_FuelPrssRegulatorStuck : Subsystem
  FAULT_08_FuelValveLeakage : Subsystem
  FAULT_09_FuelContamination : Subsystem
  FAULT_10_FuelLineBlockage : Subsystem
  FAULT_11_FuelPumpDegradation : Subsystem
  FAULT_12_FuelSupplyPressDrop : Subsystem
  FAULT_13_FGSupplyPressOscillation : Subsystem
  FAULT_16_FuelValveLeak : Subsystem
  Manual Switch{1..8} (8 alike) : ManualSwitch
  Prss_FG_Aftr_MCV_PT204_kPa : ToWorkspace  VariableName=Prss_FG_Aftr_MCV_PT204_kPa  SampleTime=0.2
  Subsystem1 : Subsystem
  FG Temp (oC) : Outport
  FG Flow @bur (kg/s) : Outport  Port=2
  FG pr @bur (kPa) : Outport  Port=3
  FG skid inlet prss (kPa) : Outport  Port=4
  tag scope: FG_flow=global
  wires:
  Subsystem1/2(skid temp) -> CV model chamber 2/3(FG temp.)
  " Memory "/1 -> Subsystem1/3(FG flow)
  Subsystem1/1(" FG skid inlet prss") -> CV model chamber 2/2(Skid inlet prss), Prss_FG_Aftr_MCV_PT204_kPa/1, FG skid inlet prss (kPa)/1
  FG temp./1 -> Subsystem1/2(FG temp.), FG Temp (oC)/1
  CV model chamber 2/1(FG pr @bur) -> FG pr @bur (kPa)/1
  FG CV pos (%) chmb1/1 -> CV model chamber 2/1(FG valve pos.)
  FAULT_16_FuelValveLeak/1(Out1) -> Manual Switch7/1
  CV model chamber 2/2(FG flow) -> Manual Switch7/2, FAULT_16_FuelValveLeak/1(FG flow)
  FAULT_09_FuelContamination/1(Out1) -> Manual Switch1/1
  FAULT_10_FuelLineBlockage/1(Out1) -> Manual Switch2/1
  Manual Switch2/1 -> FG Flow @bur (kg/s)/1, " Memory "/1, [FG_flow]
  Manual Switch7/1 -> Manual Switch1/2, FAULT_09_FuelContamination/1(In1)
  FAULT_13_FGSupplyPressOscillation/1(Out1) -> Manual Switch3/1
  FAULT_12_FuelSupplyPressDrop/1(Out1) -> Manual Switch4/1
  FAULT_11_FuelPumpDegradation/1(Out1) -> Manual Switch5/1
  FAULT_07_FuelPrssRegulatorStuck/1(Out1) -> Manual Switch6/1
  Manual Switch3/1 -> Subsystem1/1(gas prss)
  Manual Switch4/1 -> Manual Switch3/2, FAULT_13_FGSupplyPressOscillation/1(In1)
  Manual Switch5/1 -> Manual Switch4/2, FAULT_12_FuelSupplyPressDrop/1(In1)
  Manual Switch6/1 -> Manual Switch5/2, FAULT_11_FuelPumpDegradation/1(In1)
  main FG line prss/1 -> Manual Switch6/2, FAULT_07_FuelPrssRegulatorStuck/1(main FG line prss)
  Manual Switch1/1 -> Manual Switch8/2, FAULT_08_FuelValveLeakage/1(In1)
  FAULT_08_FuelValveLeakage/1(Out1) -> Manual Switch8/1
  Manual Switch8/1 -> Manual Switch2/2, FAULT_10_FuelLineBlockage/1(In1)

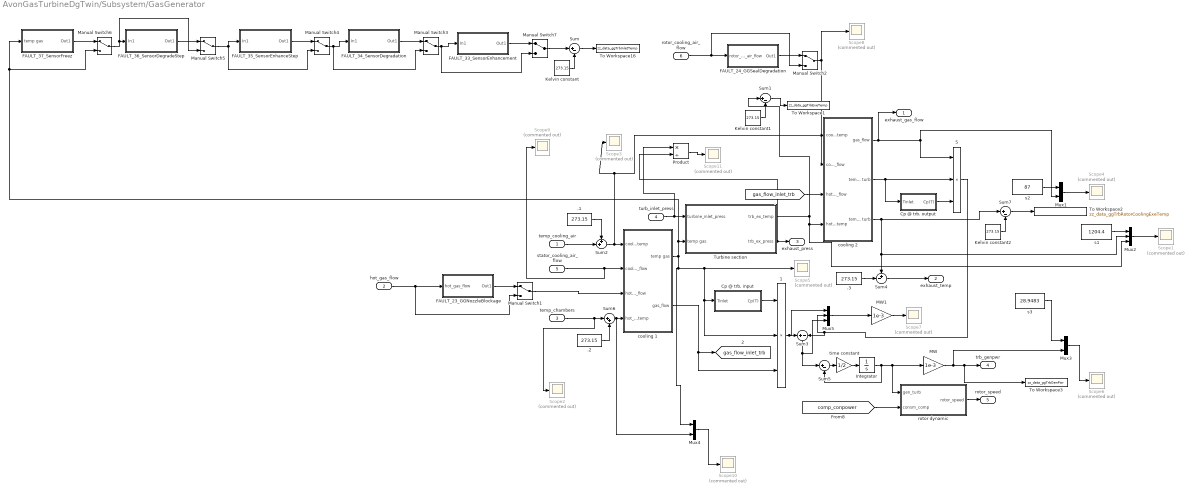
== system AvonGasTurbineDgTwin/Subsystem/GasGenerator ==
  temp_cooling_air : Inport
  hot_gas_flow : Inport  Port=2
  temp_chambers : Inport  Port=3
  turb_inlet_press : Inport  Port=4
  stator_cooling_air_flow : Inport  Port=5
  rotor_cooling_air_flow : Inport  Port=6
  "    .1" : Constant  Value=273.15
  "    .2" : Constant  Value=273.15
  "    .3" : Constant  Value=273.15
  " 1" : Product  Inputs=3  RndMeth=Zero
  " 5" : Product  Inputs=3  RndMeth=Zero
  Cp @ trb. input : Subsystem
  Cp @ trb. output : Subsystem
  FAULT_23_GGNozzleBlockage : Subsystem
  FAULT_24_GGSealDegradation : Subsystem
  FAULT_33_SensorEnhancement : Subsystem
  FAULT_34_SensorDegradation : Subsystem
  FAULT_35_SensorEnhanceStep : Subsystem
  FAULT_36_SensorDegradeStep : Subsystem
  FAULT_37_SensorFreez : Subsystem
  Integrator : Integrator  InitialCondition=13500  LimitOutput=on  UpperSaturationLimit=34000  LowerSaturationLimit=10
  Kelvin constant : Constant  Value=273.15
  Kelvin constant1 : Constant  Value=273.15
  Kelvin constant2 : Constant  Value=273.15
  MW : Gain  Gain=1e-3
  MW1 : Gain  Gain=1e-3
  Manual Switch{1..7} (7 alike) : ManualSwitch
  Mux1 : Mux  Inputs=2
  Mux2 : Mux  Inputs=3
  Mux3 : Mux  Inputs=2
  Mux4 : Mux  Inputs=2
  Mux5 : Mux  Inputs=3
  Product : Product  Inputs=*/
  Scope{1..11} (11 alike) : Scope  Commented=on
  Sum{,1,5,7} (4 alike) : Sum  Inputs=|+-
  Sum2 : Sum  Inputs=++|
  Sum3 : Sum  Inputs=+-
  Sum4 : Sum  Inputs=+-|
  Sum6 : Sum  Inputs=|++
  To Workspace1 : ToWorkspace  VariableName=zz_data_ggTrbExeTemp  SampleTime=0.2
  To Workspace16 : ToWorkspace  VariableName=zz_data_ggTrbInletTemp  SampleTime=0.2
  To Workspace2 : ToWorkspace  VariableName=zz_data_ggTrbRotorCoolingExeTemp  SampleTime=0.2
  To Workspace3 : ToWorkspace  VariableName=zz_data_ggTrbGenPwr  SampleTime=0.2
  Turbine section : Subsystem
  cooling 1 : Subsystem
  cooling 2 : Subsystem
  "rotor dynamic " : Subsystem
  s1 : Constant  Value=1204.4
  s2 : Constant  Value=87
  s3 : Constant  Value=28.9483
  time constant : Gain  Gain=1/2
  exhaust_gas_flow : Outport
  exhaust_temp : Outport  Port=2
  exhaust_press : Outport  Port=3
  trb_genpwr : Outport  Port=4
  rotor_speed : Outport  Port=5
  tag scope: gas_flow_inlet_trb=global
  wires:
  Sum2/1 -> cooling 1/1(cooling_air_temp), cooling 2/1(cooling_air_temp), Scope3/1
  " 1"/1 -> Mux5/1, Sum3/1
  Sum5/1 -> time constant/1
  time constant/1 -> Integrator/1
  [gas_flow_inlet_trb] -> cooling 2/3(hot_gas_flow)
  Cp @ trb. input/1(Cp(T)) -> " 1"/1
  Turbine section/1(trb_ex_temp) -> Sum1/1, Mux2/3, cooling 2/4(hot_gas_temp)
  cooling 2/3(temp exh turb) -> Sum7/1, Mux2/2, Sum4/1
  Cp @ trb. output/1(Cp(T)) -> " 5"/3
  " 5"/1 -> Sum3/2, Mux5/2
  cooling 1/2(gas_flow) -> " 1"/3, [gas_flow_inlet_trb]
  Sum3/1 -> Mux5/3, Sum5/1
  Mux1/1 -> Scope4/1
  s2/1 -> Mux1/1
  cooling 2/1(gas_flow) -> " 5"/1, Mux1/2, exhaust_gas_flow/1
  Mux2/1 -> Scope1/1
  s1/1 -> Mux2/1
  "    .1"/1 -> Sum2/1
  temp_cooling_air/1 -> Sum2/2
  "    .2"/1 -> Sum6/2
  temp_chambers/1 -> Scope2/1, Sum6/1
  Sum4/1 -> exhaust_temp/1
  "    .3"/1 -> Sum4/2
  turb_inlet_press/1 -> Product/1, Turbine section/1(turbine_inlet_press)
  Mux3/1 -> Scope6/1
  s3/1 -> Mux3/1
  Integrator/1 -> "rotor dynamic "/1(gen_turb), MW/1, Sum5/2
  cooling 2/2(temp turb) -> Cp @ trb. output/1(Tinlet), " 5"/2
  Turbine section/2(trb_ex_press) -> exhaust_press/1, Product/2
  MW/1 -> Mux3/2, To Workspace3/1, trb_genpwr/1
  [comp_conpower] -> "rotor dynamic "/2(consm_comp)
  "rotor dynamic "/1(rotor_speed) -> rotor_speed/1
  stator_cooling_air_flow/1 -> cooling 1/2(cooling_air_flow), Scope9/1
  Mux4/1 -> Scope10/1
  cooling 1/1(temp gas) -> FAULT_37_SensorFreez/1(temp gas), Manual Switch6/2, Turbine section/2(temp gas), Cp @ trb. input/1(Tinlet), " 1"/2, Scope5/1, Mux4/1
  Sum6/1 -> Mux4/2, cooling 1/4(hot_gas_temp)
  Mux5/1 -> MW1/1
  MW1/1 -> Scope7/1
  Product/1 -> Scope11/1
  FAULT_23_GGNozzleBlockage/1(Out1) -> Manual Switch1/1
  Manual Switch1/1 -> cooling 1/3(hot_gas_flow)
  hot_gas_flow/1 -> Manual Switch1/2, FAULT_23_GGNozzleBlockage/1(hot_gas_flow)
  FAULT_24_GGSealDegradation/1(Out1) -> Manual Switch2/1
  rotor_cooling_air_flow/1 -> Manual Switch2/2, FAULT_24_GGSealDegradation/1(rotor_cooling_air_flow)
  Manual Switch2/1 -> cooling 2/2(cooling_air_flow), Scope8/1
  FAULT_33_SensorEnhancement/1(Out1) -> Manual Switch7/1
  FAULT_34_SensorDegradation/1(Out1) -> Manual Switch3/1
  FAULT_35_SensorEnhanceStep/1(Out1) -> Manual Switch4/1
  FAULT_36_SensorDegradeStep/1(Out1) -> Manual Switch5/1
  FAULT_37_SensorFreez/1(Out1) -> Manual Switch6/1
  Manual Switch3/1 -> Manual Switch7/2, FAULT_33_SensorEnhancement/1(In1)
  Manual Switch4/1 -> Manual Switch3/2, FAULT_34_SensorDegradation/1(In1)
  Manual Switch5/1 -> Manual Switch4/2, FAULT_35_SensorEnhanceStep/1(In1)
  Manual Switch6/1 -> Manual Switch5/2, FAULT_36_SensorDegradeStep/1(In1)
  Kelvin constant/1 -> Sum/2
  Manual Switch7/1 -> Sum/1
  Sum/1 -> To Workspace16/1
  Kelvin constant1/1 -> Sum1/2
  Sum1/1 -> To Workspace1/1
  Kelvin constant2/1 -> Sum7/2
  Sum7/1 -> To Workspace2/1

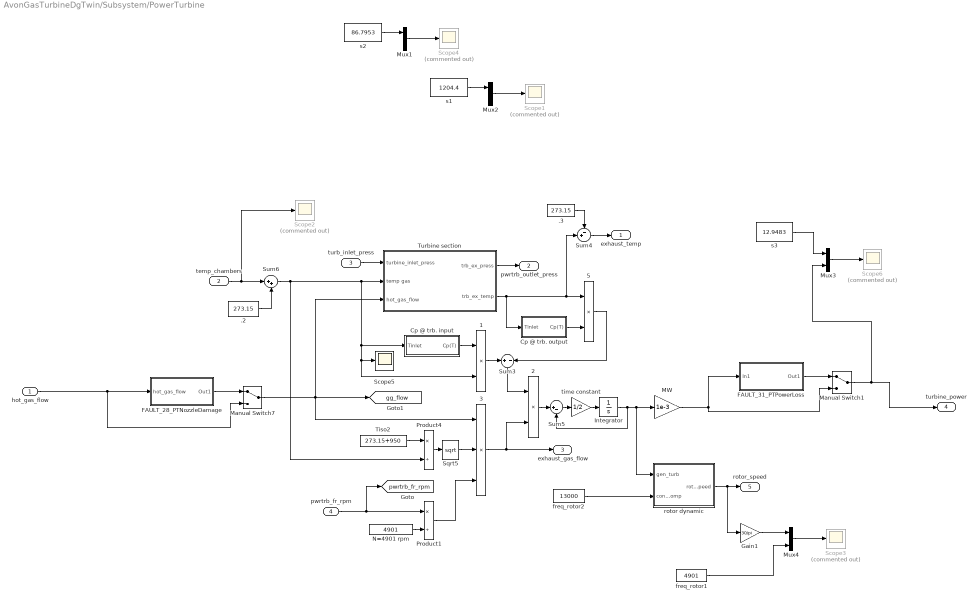
== system AvonGasTurbineDgTwin/Subsystem/PowerTurbine ==
  hot_gas_flow : Inport
  temp_chambers : Inport  Port=2
  turb_inlet_press : Inport  Port=3
  pwrtrb_fr_rpm : Inport  Port=4
  "    .2" : Constant  Value=273.15
  "    .3" : Constant  Value=273.15
  " 1" : Product  RndMeth=Zero
  " 2" : Product  RndMeth=Zero
  " 3" : Product  Inputs=3  RndMeth=Zero
  " 5" : Product  RndMeth=Zero
  Cp @ trb. input : Subsystem
  Cp @ trb. output : Subsystem
  FAULT_28_PTNozzleDamage : Subsystem
  FAULT_31_PTPowerLoss : Subsystem
  Gain1 : Gain  Gain=30/pi
  Integrator : Integrator  InitialCondition=13000  LimitOutput=on  UpperSaturationLimit=20000  LowerSaturationLimit=1
  MW : Gain  Gain=1e-3
  Manual Switch1 : ManualSwitch
  Manual Switch7 : ManualSwitch
  Mux1 : Mux  Inputs=2
  Mux2 : Mux  Inputs=3
  Mux3 : Mux  Inputs=2
  Mux4 : Mux  Inputs=2
  N=4901 rpm : Constant  Value=4901
  Product1 : Product  Inputs=*/  RndMeth=Zero
  Product4 : Product  Inputs=*/  RndMeth=Zero
  Scope{1..4,6} (5 alike) : Scope  Commented=on
  Scope5 : Scope
  Sqrt5 : Sqrt
  Sum3 : Sum  Inputs=+-
  Sum4 : Sum  Inputs=-+|
  Sum5 : Sum  Inputs=|+-
  Sum6 : Sum  Inputs=|++
  Tiso2 : Constant  Value=273.15+950
  Turbine section : Subsystem
  freq_rotor1 : Constant  Value=4901
  freq_rotor2 : Constant  Value=13000
  rotor dynamic : Subsystem
  s1 : Constant  Value=1204.4
  s2 : Constant  Value=86.7953
  s3 : Constant  Value=12.9483
  time constant : Gain  Gain=1/2
  exhaust_temp : Outport
  pwrtrb_outlet_press : Outport  Port=2
  exhaust_gas_flow : Outport  Port=3
  turbine_power : Outport  Port=4
  rotor_speed : Outport  Port=5
  tag scope: gg_flow=global, pwrtrb_fr_rpm=global
  wires:
  Turbine section/2(trb_ex_temp) -> " 5"/1, Sum4/2, Cp @ trb. output/1(Tinlet)
  s3/1 -> Mux3/1
  Mux3/1 -> Scope6/1
  turb_inlet_press/1 -> Turbine section/1(turbine_inlet_press)
  "    .3"/1 -> Sum4/1
  Sum4/1 -> exhaust_temp/1
  temp_chambers/1 -> Scope2/1, Sum6/1
  "    .2"/1 -> Sum6/2
  s1/1 -> Mux2/1
  Mux2/1 -> Scope1/1
  s2/1 -> Mux1/1
  Mux1/1 -> Scope4/1
  " 2"/1 -> Sum5/1
  " 5"/1 -> Sum3/2
  Cp @ trb. output/1(Cp(T)) -> " 5"/2
  Cp @ trb. input/1(Cp(T)) -> " 1"/1
  time constant/1 -> Integrator/1
  Sum5/1 -> time constant/1
  " 1"/1 -> Sum3/1
  Sum3/1 -> " 2"/1
  Tiso2/1 -> Product4/1
  Sum6/1 -> Product4/2, Cp @ trb. input/1(Tinlet), " 1"/2, Scope5/1, Turbine section/2(temp gas)
  Product4/1 -> Sqrt5/1
  N=4901 rpm/1 -> Product1/2
  pwrtrb_fr_rpm/1 -> [pwrtrb_fr_rpm], Product1/1
  Product1/1 -> " 3"/3
  Sqrt5/1 -> " 3"/2
  " 3"/1 -> exhaust_gas_flow/1, " 2"/2
  Turbine section/1(trb_ex_press) -> pwrtrb_outlet_press/1
  rotor dynamic/1(rotor_speed) -> Gain1/1, rotor_speed/1
  Integrator/1 -> Sum5/2, MW/1, rotor dynamic/1(gen_turb)
  Mux4/1 -> Scope3/1
  freq_rotor1/1 -> Mux4/2
  Gain1/1 -> Mux4/1
  freq_rotor2/1 -> rotor dynamic/2(consm_comp)
  FAULT_28_PTNozzleDamage/1(Out1) -> Manual Switch7/1
  Manual Switch7/1 -> " 3"/1, Turbine section/3(hot_gas_flow), [gg_flow]
  hot_gas_flow/1 -> Manual Switch7/2, FAULT_28_PTNozzleDamage/1(hot_gas_flow)
  FAULT_31_PTPowerLoss/1(Out1) -> Manual Switch1/1
  MW/1 -> FAULT_31_PTPowerLoss/1(In1), Manual Switch1/2
  Manual Switch1/1 -> Mux3/2, turbine_power/1

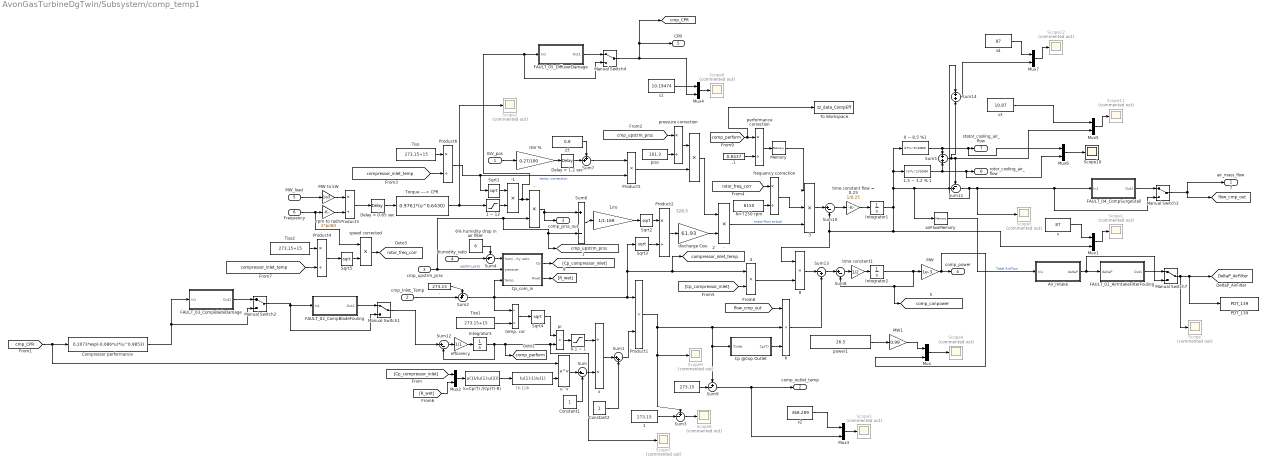
== system AvonGasTurbineDgTwin/Subsystem/comp_temp1 ==
  note: (k-1)/k
  note: 328.5
  IGV_pos : Inport
  cmp_Inlet_Temp : Inport  Port=2
  cmp_upstrm_prss : Inport  Port=3
  humidity_ratio : Inport  Port=4
  MW_load : Inport  Port=5
  Frequency : Inport  Port=6
  " " : Fcn  Expr=(u(1)-1)/u(1)
  "    " : Constant  Value=273.15
  "     " : Product  RndMeth=Zero
  "    1" : Constant  Value=273.15
  " 1.5 ~ 3.2 % 1" : Fcn  Expr=(17*u^2)/16000  SampleTime=1
  " 3" : Product  Inputs=3  RndMeth=Zero
  " 4" : Product  RndMeth=Zero
  " 6" : Product  Inputs=3  RndMeth=Zero
  " 8" : Product  RndMeth=Zero
  - : Product  RndMeth=Zero
  -1 : Product  RndMeth=Zero
  . : Constant  Value=273.15
  ". " : Product  RndMeth=Zero
  .1 : Constant  Value=0.8437
  0 ~ 8.5 %1 : Fcn  Expr=(17*u^2)/44000  SampleTime=1
  0.1 ~ 1 : Saturate  UpperLimit=1  LowerLimit=0.1
  1 ~ 12 : Saturate  UpperLimit=20  LowerLimit=1
  1/ro : Gain  Gain=1/1.169
  6% humidity drop in air filter : Constant  Value=6
  Air_Intake : Subsystem
  "Compressor performance " : Fcn  Expr=0.2073*exp(-0.086*u)*(u^0.9853)
  Constant1 : Constant
  Constant2 : Constant
  Cp @Cop Outlet : Subsystem
  Cp_com_in : Subsystem
  Delay = 0.85 sec : TransportDelay  DelayTime=0.85  InitialOutput=10.706
  Delay = 1.2 sec : TransportDelay  DelayTime=1.2  InitialOutput=0.27
  FAULT_01_AirIntakeFilterFouling : Subsystem
  FAULT_02_CompBladeFouling : Subsystem
  FAULT_03_CompBladeDamage : Subsystem
  FAULT_04_CompSurgeStall : Subsystem
  FAULT_05_DiffuserDamage : Subsystem
  IGV % : Gain  Gain=0.27/100
  Integrator1 : Integrator  InitialCondition=87  LimitOutput=on  UpperSaturationLimit=140  LowerSaturationLimit=1
  Integrator2 : Integrator  InitialCondition=28000  LimitOutput=on  UpperSaturationLimit=32000  LowerSaturationLimit=10
  Integrator3 : Integrator  InitialCondition=0.6  LimitOutput=on  UpperSaturationLimit=1  LowerSaturationLimit=0
  MW : Gain  Gain=1e-3
  MW to kW : Gain  Gain=1e3
  MW1 : Gain  Gain=0.99
  Manual Switch{1..4,7} (5 alike) : ManualSwitch
  Memory : Memory  InitialCondition=1.5
  Mux{,1..7} (8 alike) : Mux  Inputs=2
  N=7250 rpm : Constant  Value=8150
  PDT_139 : ToWorkspace  VariableName=PDT_139  SampleTime=0.2
  Product1 : Product  RndMeth=Zero
  Product{2..4,6} (4 alike) : Product  Inputs=*/  RndMeth=Zero
  Product5 : Product  RndMeth=Zero
  Scope{,1..9,11..12} (12 alike) : Scope  Commented=on
  Scope10 : Scope
  Sqrt{1..5} (5 alike) : Sqrt
  Sum{,8,10,12} (4 alike) : Sum  Inputs=|+-
  Sum1 : Sum  Inputs=|++
  Sum11 : Sum  Inputs=-+|
  Sum13 : Sum  Inputs=|-+
  Sum14 : Sum
  Sum2 : Sum  Inputs=++|
  Sum3 : Sum  Inputs=+-|
  Sum4 : Sum  Inputs=-+|
  Sum5 : Sum
  Sum6 : Sum  Inputs=+-
  Sum7 : Sum  Inputs=++|
  Sum9 : Sum  Inputs=+-|
  Tiso : Constant  Value=273.15+15
  Tiso1 : Constant  Value=273.15+15
  Tiso2 : Constant  Value=273.15+15
  To Workspace : ToWorkspace  VariableName=zz_data_CompEff  SampleTime=0.2
  Torque ----> CPR : Fcn  Expr=0.9761*(u^0.6430)
  airFlowMemory : Memory  InitialCondition=80
  "discharge Coe. " : Gain  Gain=61.93
  efficiency : Gain  Gain=1/1
  frequency correction : Product  Inputs=*/  RndMeth=Zero
  k=Cp(T) /(Cp(T)-R) : Fcn  Expr=u(1)/(u(1)-u(2))
  performance correction : Product  Inputs=*/  RndMeth=Zero
  piso : Constant  Value=101.3
  power1 : Constant  Value=26.5
  "pr " : Product  RndMeth=Zero
  pressure correction : Product  Inputs=*/  RndMeth=Zero
  rpm to rad/s : Gain  Gain=2*pi/60
  s : Constant  Value=87
  s1 : Constant  Value=10.19474
  s2 : Constant  Value=368.289
  s3 : Constant  Value=10.87
  s4 : Constant  Value=87
  speed corrected : Product  RndMeth=Zero
  temp. cor : Product  Inputs=/*  RndMeth=Zero
  time constant flow = 0.25 : Gain  Gain=1/0.25
  time constant1 : Gain  Gain=1/2
  u^v : Math  Operator=pow  SignedPower=on
  x : Product  Inputs=/*  RndMeth=Zero
  z3 : Constant  Value=0.8
  air_mass_flow : Outport
  comp_outlet_temp : Outport  Port=2
  comp_prss_out : Outport  Port=3
  comp_power : Outport  Port=4
  CPR : Outport  Port=5
  rotor_cooling_air_flow : Outport  Port=6
  stator_cooling_air_flow : Outport  Port=7
  tag scope: DeltaP_AirFilter=global, cmp_CPR=global, cmp_upstrm_prss=global, comp_conpower=global, comp_perform=global, compressor_inlet_temp=global, flow_cmp_out=global, rotor_freq_corr=global
  wires:
  [cmp_CPR] -> "Compressor performance "/1, u^v/1
  " "/1 -> u^v/2
  u^v/1 -> Sum/1
  Sum/1 -> x/2
  Constant2/1 -> Sum1/2
  Sum1/1 -> Product1/2
  Sum2/1 -> Cp_com_in/3(temp.), Product1/1, Sqrt3/1, [compressor_inlet_temp], " 4"/1, temp. cor/1
  x/1 -> Sum1/1
  Constant1/1 -> Sum/2
  cmp_upstrm_prss/1 -> Cp_com_in/2(pressuer), -/2, [cmp_upstrm_prss], Sum6/2  "upstrm_prss"
  cmp_Inlet_Temp/1 -> Sum2/2
  0.1 ~ 1/1 -> x/1
  k=Cp(T) /(Cp(T)-R)/1 -> " "/1
  Cp_com_in/1(Cp) -> [Cp_compressor_inlet]
  Sum4/1 -> Cp_com_in/1(humidity ratio)
  humidity_ratio/1 -> Sum4/2
  6% humidity drop in air filter/1 -> Sum4/1
  -/1 -> comp_prss_out/1, Sum6/1
  Frequency/1 -> speed corrected/1, rpm to rad/s/1
  Sum6/1 -> 1/ro/1
  1/ro/1 -> Sqrt2/1
  Sqrt3/1 -> Product2/2
  Product2/1 -> "discharge Coe. "/1
  Sqrt2/1 -> Product2/1
  IGV_pos/1 -> IGV %/1
  piso/1 -> pressure correction/2
  [cmp_upstrm_prss] -> pressure correction/1
  Product5/1 -> "     "/2
  "discharge Coe. "/1 -> ". "/2
  "     "/1 -> ". "/1
  ". "/1 -> " 3"/3  "mass flow actual"
  Product6/1 -> Product5/2, Sqrt1/1  "temp. correction"
  Tiso/1 -> Product6/1
  [compressor_inlet_temp] -> Product6/2
  pressure correction/1 -> "     "/1
  1 ~ 12/1 -> -1/2
  N=7250 rpm/1 -> frequency correction/2
  [rotor_freq_corr] -> frequency correction/1
  frequency correction/1 -> " 3"/2
  " 3"/1 -> Sum10/1
  [Cp_compressor_inlet] -> " 4"/2
  Sum10/1 -> time constant flow = 0.25/1
  time constant flow = 0.25/1 -> Integrator1/1
  " 4"/1 -> " 8"/2
  " 8"/1 -> Sum13/1
  Sqrt1/1 -> -1/1
  Sum7/1 -> Product5/1
  z3/1 -> Sum7/1
  IGV %/1 -> Delay = 1.2 sec/1
  Delay = 1.2 sec/1 -> Sum7/2
  MW_load/1 -> MW to kW/1
  Cp_com_in/2(Rwet) -> [R_wet]
  Mux2/1 -> k=Cp(T) /(Cp(T)-R)/1
  [Cp_compressor_inlet] -> Mux2/1
  [R_wet] -> Mux2/2
  Sum8/1 -> time constant1/1
  time constant1/1 -> Integrator2/1
  Sum13/1 -> Sum8/1
  ./1 -> Sum2/1
  Tiso1/1 -> temp. cor/2
  temp. cor/1 -> Sqrt4/1
  "pr "/1 -> 0.1 ~ 1/1
  Sum12/1 -> efficiency/1
  efficiency/1 -> Integrator3/1
  Sqrt4/1 -> "pr "/1
  Torque ----> CPR/1 -> Scope2/1, 1 ~ 12/1
  MW to kW/1 -> Product3/1
  rpm to rad/s/1 -> Product3/2
  Integrator3/1 -> [comp_perform], Scope7/1, "pr "/2, Sum12/2
  Integrator2/1 -> MW/1, [comp_conpower], Sum8/2
  Product1/1 -> " 6"/2, Cp @Cop Outlet/1(Tinlet), Sum9/1, Scope9/1, Sum3/1
  Cp @Cop Outlet/1(Cp(T)) -> " 6"/3
  " 6"/1 -> Sum13/2
  "    "/1 -> Sum9/2
  Tiso2/1 -> Product4/1
  [compressor_inlet_temp] -> Product4/2
  speed corrected/1 -> [rotor_freq_corr]
  Product4/1 -> Sqrt5/1
  Sqrt5/1 -> speed corrected/2
  [flow_cmp_out] -> " 6"/1
  Mux/1 -> Scope4/1
  Sum11/1 -> Sum14/1, Manual Switch3/2, FAULT_04_CompSurgeStall/1(In1), Scope5/1
  0 ~ 8.5 %1/1 -> Sum5/1, Mux6/1, stator_cooling_air_flow/1
  Integrator1/1 -> Mux1/2, " 8"/1, Sum10/2, airFlowMemory/1, Sum11/2, " 1.5 ~ 3.2 % 1"/1, 0 ~ 8.5 %1/1
  Mux1/1 -> Scope1/1
  s/1 -> Mux1/1
  Product3/1 -> Delay = 0.85 sec/1
  Delay = 0.85 sec/1 -> Torque ----> CPR/1
  power1/1 -> MW1/1
  Mux3/1 -> Scope3/1
  s2/1 -> Mux3/1
  MW/1 -> Mux/2, comp_power/1
  Mux4/1 -> Scope6/1
  s1/1 -> Mux4/1
  -1/1 -> -/1, Manual Switch4/2, FAULT_05_DiffuserDamage/1(In1)
  Sum9/1 -> Mux3/2, comp_outlet_temp/1
  "    1"/1 -> Sum3/2
  Sum3/1 -> Scope8/1
  MW1/1 -> Mux/1
  Sum5/1 -> Sum14/2, Sum11/1, Mux5/2
  Mux5/1 -> Scope11/1
  s3/1 -> Mux5/1
  Mux6/1 -> Scope10/1
  " 1.5 ~ 3.2 % 1"/1 -> Sum5/2, Mux6/2, rotor_cooling_air_flow/1
  Sum14/1 -> Mux7/2
  Mux7/1 -> Scope12/1
  s4/1 -> Mux7/1
  performance correction/1 -> Memory/1
  .1/1 -> performance correction/2
  [comp_perform] -> To Workspace/1, performance correction/1
  Memory/1 -> " 3"/1
  FAULT_02_CompBladeFouling/1(Out1) -> Manual Switch1/1
  "Compressor performance "/1 -> FAULT_03_CompBladeDamage/1(In1), Manual Switch2/2
  Manual Switch1/1 -> Sum12/1
  FAULT_03_CompBladeDamage/1(Out1) -> Manual Switch2/1
  Manual Switch2/1 -> Manual Switch1/2, FAULT_02_CompBladeFouling/1(In1)
  FAULT_04_CompSurgeStall/1(Out1) -> Manual Switch3/1
  Manual Switch3/1 -> [flow_cmp_out], air_mass_flow/1
  FAULT_05_DiffuserDamage/1(Out1) -> Manual Switch4/1
  Manual Switch4/1 -> Mux4/2, CPR/1, [cmp_CPR]
  airFlowMemory/1 -> Air_Intake/1(In1)  "Total AirFlow"
  FAULT_01_AirIntakeFilterFouling/1(Out1) -> Manual Switch7/1
  Air_Intake/1(deltaP) -> Manual Switch7/2, FAULT_01_AirIntakeFilterFouling/1(deltaP)
  Manual Switch7/1 -> Scope/1, PDT_139/1, [DeltaP_AirFilter]

== system AvonGasTurbineDgTwin/Subsystem2/FAULT_42_ControlLoopOscillation ==
  In1 : Inport
  FAULT_42_multiplier : FromWorkspace  VariableName=FAULT_42_multiplier  SampleTime=-1
  Mux : Mux  Inputs=2
  Product : Product
  Scope{,1..3} (4 alike) : Scope  Commented=on
  Out1 : Outport
  wires:
  FAULT_42_multiplier/1 -> Product/1, Scope/1
  In1/1 -> Scope1/1, Mux/2, Product/2
  Product/1 -> Mux/1, Scope2/1, Out1/1
  Mux/1 -> Scope3/1

== system AvonGasTurbineDgTwin/Subsystem/Combustor1/FAULT_16_CombLinerDamage ==
  air_flow : Inport
  FAULT_16_multiplier : FromWorkspace  VariableName=FAULT_16_multiplier  SampleTime=-1
  Mux : Mux  Inputs=2
  Product : Product
  Scope{,1..3} (4 alike) : Scope  Commented=on
  Out1 : Outport
  wires:
  FAULT_16_multiplier/1 -> Product/1, Scope/1
  air_flow/1 -> Scope1/1, Mux/2, Product/2
  Product/1 -> Mux/1, Scope2/1, Out1/1
  Mux/1 -> Scope3/1

== system AvonGasTurbineDgTwin/Subsystem/Combustor1/FAULT_17_FuelNozzleClogging ==
  FG flow : Inport
  FAULT_17_multiplier : FromWorkspace  VariableName=FAULT_17_multiplier  SampleTime=-1
  Mux : Mux  Inputs=2
  Product : Product
  Scope{,1..3} (4 alike) : Scope  Commented=on
  Out1 : Outport
  wires:
  FAULT_17_multiplier/1 -> Product/1, Scope/1
  FG flow/1 -> Scope1/1, Mux/2, Product/2
  Product/1 -> Mux/1, Scope2/1, Out1/1
  Mux/1 -> Scope3/1

== system AvonGasTurbineDgTwin/Subsystem/Combustor1/FAULT_18_CombustionFlameOscillation ==
  temp chamber 1 : Inport
  FAULT_18_multiplier : FromWorkspace  VariableName=FAULT_18_multiplier  SampleTime=-1
  Mux : Mux  Inputs=2
  Product : Product
  Scope{,1..3} (4 alike) : Scope  Commented=on
  Out1 : Outport
  wires:
  FAULT_18_multiplier/1 -> Product/1, Scope/1
  temp chamber 1/1 -> Scope1/1, Mux/2, Product/2
  Product/1 -> Mux/1, Scope2/1, Out1/1
  Mux/1 -> Scope3/1

== system AvonGasTurbineDgTwin/Subsystem/Combustor1/FAULT_19_CombustionInstability ==
  In1 : Inport
  FAULT_19_multiplier : FromWorkspace  VariableName=FAULT_19_multiplier  SampleTime=-1
  Mux : Mux  Inputs=2
  Product : Product
  Scope{,1..3} (4 alike) : Scope  Commented=on
  Out1 : Outport
  wires:
  FAULT_19_multiplier/1 -> Product/1, Scope/1
  In1/1 -> Scope1/1, Mux/2, Product/2
  Product/1 -> Mux/1, Scope2/1, Out1/1
  Mux/1 -> Scope3/1

== system AvonGasTurbineDgTwin/Subsystem/Combustor1/FAULT_20_HotGasPathTempIncrease ==
  In1 : Inport
  FAULT_20_multiplier : FromWorkspace  VariableName=FAULT_20_multiplier  SampleTime=-1
  Mux : Mux  Inputs=2
  Product : Product
  Scope{,1..3} (4 alike) : Scope  Commented=on
  Out1 : Outport
  wires:
  FAULT_20_multiplier/1 -> Product/1, Scope/1
  In1/1 -> Scope1/1, Mux/2, Product/2
  Product/1 -> Mux/1, Scope2/1, Out1/1
  Mux/1 -> Scope3/1
